simulink model "lab"  (R2024b)
settings: Solver=ode4  StartTime=0.0  StopTime=20.0  FixedStep=0.01  RelTol=1e-3
values from neighbouring files (symbols this model uses):
  A = [0 0 0; 1 0 -1; 0 1 2]    [main.m]
  B = [0 -1; 1 0; 0 1]    [main.m]
  C = [1 0 1]    [main.m]
  F = f0 + g * fT    [main.m]
  g = randn(m, 1)    [main.m]
settings Model: Creator=rober  LastModifiedBy=rober

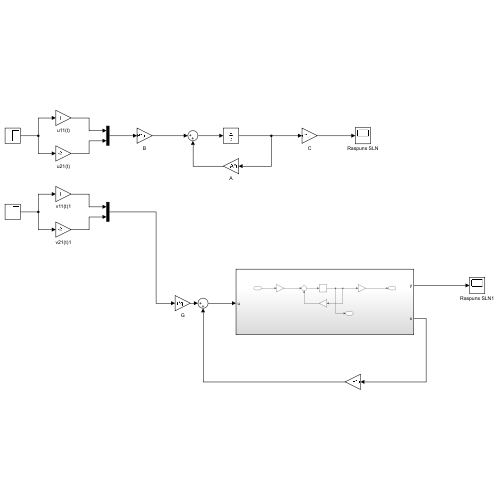
[thumbnail: Simulink's stored preview of the top-level diagram]
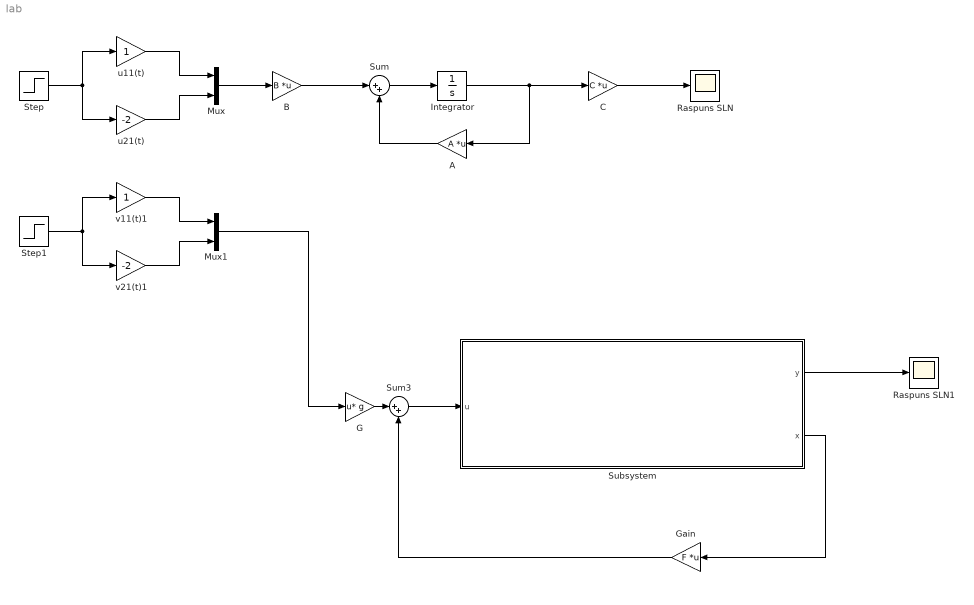
== system lab ==
  A : Gain  Gain=A  Multiplication=Matrix(K*u)
  B : Gain  Gain=B  Multiplication=Matrix(K*u)
  C : Gain  Gain=C  Multiplication=Matrix(K*u)
  G : Gain  Gain=g  Multiplication=Matrix(u*K)
  Gain : Gain  Gain=F  Multiplication=Matrix(K*u)
  Integrator : Integrator
  Mux : Mux  Inputs=2
  Mux1 : Mux  Inputs=2
  Raspuns SLN : Scope
  Raspuns SLN1 : Scope
  Step : Step  SampleTime=0
  Step1 : Step  SampleTime=0
  Subsystem : Subsystem
  Sum : Sum  Inputs=|++
  Sum3 : Sum  Inputs=|++
  u11(t) : Gain
  u21(t) : Gain  Gain=-2
  v11(t)1 : Gain
  v21(t)1 : Gain  Gain=-2
  wires:
  Step/1 -> u11(t)/1, u21(t)/1
  u11(t)/1 -> Mux/1
  u21(t)/1 -> Mux/2
  Mux/1 -> B/1
  B/1 -> Sum/1
  A/1 -> Sum/2
  Sum/1 -> Integrator/1
  Integrator/1 -> A/1, C/1
  C/1 -> Raspuns SLN/1
  Mux1/1 -> G/1
  v21(t)1/1 -> Mux1/2
  Step1/1 -> v11(t)1/1, v21(t)1/1
  v11(t)1/1 -> Mux1/1
  Sum3/1 -> Subsystem/1(u)
  G/1 -> Sum3/1
  Subsystem/1(y) -> Raspuns SLN1/1
  Subsystem/2(x) -> Gain/1
  Gain/1 -> Sum3/2

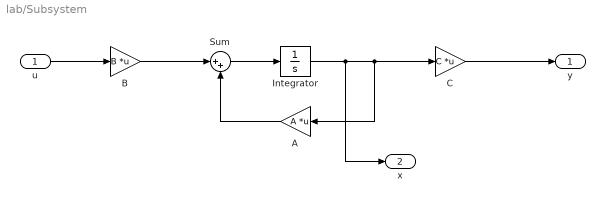
== system lab/Subsystem ==
  u : Inport
  A : Gain  Gain=A  Multiplication=Matrix(K*u)
  B : Gain  Gain=B  Multiplication=Matrix(K*u)
  C : Gain  Gain=C  Multiplication=Matrix(K*u)
  Integrator : Integrator
  Sum : Sum  Inputs=|++
  y : Outport
  x : Outport  Port=2
  wires:
  Integrator/1 -> x/1, A/1, C/1
  B/1 -> Sum/1
  u/1 -> B/1
  A/1 -> Sum/2
  Sum/1 -> Integrator/1
  C/1 -> y/1
